simulink model "Engine_Plant_Live"  (R2026b)
settings: Solver=ode1  StartTime=0  StopTime=simcfg.stop_time  FixedStep=0.001
undefined symbols (not defined in the file): constants, ident, init, limits, simcfg
settings Model: Creator=leont  LastModifiedBy=williamvandevoir
settings DataIOCC: ExternalInput=data.ext_in  SaveOutput=off

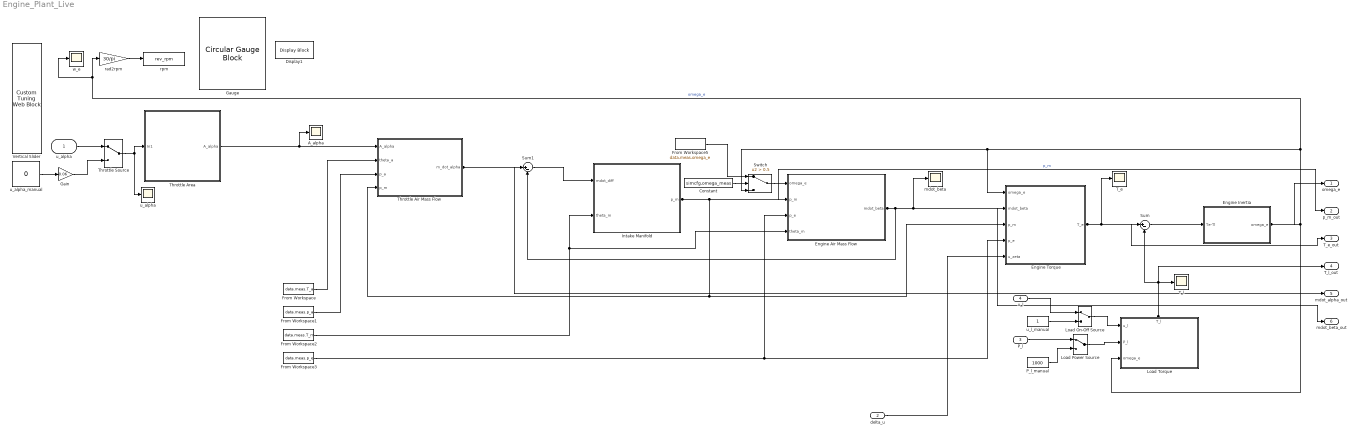
== system Engine_Plant_Live ==
  u_alpha : Inport
  delta_u : Inport  Port=2
  P_l : Inport  Port=3
  u_l : Inport  Port=4
  A_alpha : Scope
      settings: DataLoggingVariableName=ScopeData4
  Constant : Constant  Value=simcfg.omega_meas
  Display1 : DisplayBlock  LabelPosition=Hide  Format=Integer  Transparency=1  GridColor=[0.502, 0.502, 0.502]
  Engine Air Mass Flow : Subsystem
  Engine Inertia : Subsystem
  Engine Torque : Subsystem
  From Workspace : FromWorkspace  VariableName=data.meas.T_a
  From Workspace1 : FromWorkspace  VariableName=data.meas.p_a
  From Workspace2 : FromWorkspace  VariableName=data.meas.T_m
  From Workspace3 : FromWorkspace  VariableName=data.meas.p_e
  From Workspace5 : FromWorkspace  VariableName=data.meas.omega_e
  Gain : Gain  Gain=0.06
  Gauge : CircularGaugeBlock  ScaleMax=5000  FontColor=[0.0, 0.0, 0.0]
  Intake Manifold : Subsystem  Description=Adapted from Intake Manifold Exercise (pressure dynamics only): dp_m/dt = R*theta_m/Vm*(mdot_alpha - mdot_beta). One state; theta_m is an input; R instead of kappa*R.
  Load On-Off Source : ManualSwitch
  Load Power Source : ManualSwitch
  Load Torque : Subsystem
      settings: PortSchema="{\"entries\":[{\"content\":{\"sides\":[{\"content\":{\"connectorIds\":[\"In1\",\"In2\",\"In3\"]},\"type\":\"ConnectorPlacement.EquallySpacedRectSide\",\"uuid\":\"10634893-d67a-46d0-98c2-3f8faa6507dc\"},{\"content\":{\"side\":\"RIGHT\"},\"type\":\"ConnectorPlacement.EquallySpacedRectSide\",\"uuid\":\"a9acb188-8b21-47a2-8013-48c002daa6a2\"},{\"content\":{\"connectorIds\":[\"Out1\"],\"side\":\"TOP\"},\"type\":\"ConnectorPlacement.EquallySpacedRectSide\",\"uuid\":\"c0cacd4e-ae12-4b4a-9868-6a43ffe5219b\"}]},\"type\":\"ConnectorPlacement.EquallySpacedConnector\",\"uuid\":\"1dbc25fc-6040-4af1-8208-de8f0fac67f2\"}],\"packageUris\":[\"http://schema.mathworks.com/mf0/Connector/R2020b\"],\"version\":\"1.0\"}"
  P_l_manual : Constant  Value=1000
  Sum : Sum  Inputs=|+-
  Sum1 : Sum  Inputs=|+-
  Switch : Switch  Criteria=u2 > Threshold  Threshold=0.5  SaturateOnIntegerOverflow=off  InputSameDT=off
  T_e : Scope
      settings: ActiveDisplayYMinimum=-24.090812904473726  ActiveDisplayYMaximum=17.370443961385767
  T_l : Scope
      settings: ActiveDisplayYMinimum=61.428571428571431  ActiveDisplayYMaximum=81.428571428571431
  Throttle Air Mass Flow : Subsystem
  Throttle Area : Subsystem
  Throttle Source : ManualSwitch
  Vertical Slider : CustomTuningWebBlock  LabelPosition=Hide  ShowInitialText=on  Configuration="{\"components\":[{\"name\":\"LinearScaleComponent\",\"settings\":{\"bounds\":{\"max\":100,\"min\":0,\"tickInterval\":\"auto\"},\"internalTickHeightScaleFactor\":0.5,\"labelColor\":[255,255,200],\"labelFont\":{\"font\":\"Arial\",\"fontSize\":12},\"labelOffset\":0.05,\"labelTransparency\":1,\"needleImage\":{\"size\":[596,842],\"src\":\"data:image\\/svg+xml;base64,PD94bWwgdmVyc2lvbj0iMS4wIiBlbmNvZGluZz0idXRmLTgiPz4NCjwhLS0gR2VuZXJhdG9yOiBBZG9iZSBJbGx1c3RyYXRvciAyNS4wLjAsIFNWRyBFeHBvcnQgUGx1Zy1JbiAuIFNWRyBWZXJzaW9uOiA2LjAwIEJ1aWxkIDApICAtLT4NCjxzdmcgdmVyc2lvbj0iMS4xIg0KCSBpZD0ic3ZnOCIgeG1sbnM6Y2M9Imh0dHA6Ly9jcmVhdGl2ZWNvbW1vbnMub3JnL25zIyIgeG1sbnM6ZGM9Imh0dHA6Ly9wdXJsLm9yZy9kYy9lbGVtZW50cy8xLjEvIiB4bWxuczppbmtzY2FwZT0iaHR0cDovL3d3dy5pbmtzY2FwZS5vcmcvbmFtZXNw ...(+2420 chars)\",\"srcOrientation\":\"horizontal\"},\"needleOffset\":[0.0642123287671233,-0.8044596912521441],\"needleSize\":{\"height\":0.07668067226890757,\"width\":0.4337797619047619},\"position\":[0.03623949579831933,0.2829861111111111,0.6088789682539683,0.9196428571428571],\"referencePoint\":\"auto\",\"scaleColors\":[],\"scaleColorsSize\":0.2,\"scaleDirection\":\"BT\",\"showLabels\":1,\"showMinorTicks\":0,\"showSpanLine\":1,\"showTicks\":1,\"tickColor\":[252,252,197],\"tickTransparency\":1,\"valueBarColor\":[0,114,189],\"valueBarOffset\":-0.27,\"valueBarSize\":0.1,\"valueBarTransparency\":1}},{\"name\":\"BackgroundImageComponent\",\"settings\":{\"image\":{\"size\":[380,101],\"src\":\"data:image\\/svg+xml;base64,PHN2ZyB4bWxucz0iaHR0cDovL3d3dy53My5vcmcvMjAwMC9zdmciIHhtbG5zOnhsaW5rPSJodHRwOi8vd3d3LnczLm9yZy8xOTk5L3hsaW5rIiB2aWV3Qm94PSIwIDAgMzgwIDEwMSI+PGRlZnM+PHN0eWxlPi5jbHMtMXtmaWxsOiMwMDJiNDI7fS5jbHMtMntmaWxsOiM0MjcwODI7fS5jbHMtM3tmaWxsOnVybCgjcmFkaWFsLWdyYWRpZW50KTt9LmNscy00e2ZpbGw6I2M4YzhjODtzdHJva2U6IzAwMDt9PC9zdHlsZT48cmFkaWFsR3JhZGllbnQgaWQ9InJhZGlhbC1ncmFkaWVudCIgY3g9IjE5MCIgY3k9IjUwLjUiIHI9IjI2OS4yMSIgZ3JhZGllbnRVbml0cz0idXNlclNwYWNlT25Vc2UiPjxzdG9wIG9mZnNldD0iMC4wMSIgc3RvcC1jb2xvcj0iIzNlNGY1OCIvPjxzdG9wIG9mZnNldD0iMC4wNiIgc3RvcC1jb2xvcj0iIzQ0NTc2MSIvPjxzdG9wIG9mZnNldD0iMC4xNSIgc3RvcC1jb2xvcj0iIzU1NmE3NiIvPjxzdG9wIG9mZnNldD0iMC4yNSIgc3RvcC1jb2xvcj0iIzZkODg5NSIvPjxzdG9wIG9mZnNldD0iMC4zOCIgc3RvcC1jb2xvcj0iIzhmYjJjMyIvPjxzdG9wIG9mZnNldD0iMC41MiIgc3RvcC1jb2xvcj0iI2I2ZTRmYSIvPjxzdG9wIG9mZnNldD0iMSIgc3RvcC1jb2xvcj0iIzE1NDY1NyIvPjwvcmFkaWFsR3JhZGllbnQ+PC9kZWZzPjxnIGlkPSJmcmFtZSI+PGcgaWQ9IkxheWVyXzIiIGRhdGEtbmFtZT0iTGF5ZXIgMiI+PGcgaWQ9IkxheWVyXzEtMiIgZGF0YS1uYW1lPSJMYXllciAxLTIiPjxyZWN0IGlkPSJyZWN0MTAzNiIgY2xhc3M9ImNscy0xIiB4PSIxMSIgeT0iMTEiIHdpZHRoPSIzNTgiIGhlaWdodD0iNzkiLz48cGF0aCBpZD0icGF0aDEwMzgiIGNsYXNzPSJjbHMtMiIgZD0iTTgsOFY5M0gzNzJWOFpNMzY5LDkwSDExVjExSDM2OVoiLz48cGF0aCBpZD0icGF0aDEwNDAiIGNsYXNzPSJjbHMtMyIgZD0iTTAsMFYxMDFIMzgwVjBaTTM3Miw5M0g4VjhIMzcyWiIvPjwvZz48L2c+PC9nPjxnIGlkPSJ0cmFjayI+PHBhdGggaWQ9InJlY3QxNjExIiBjbGFzcz0iY2xzLTQiIGQ9Ik0zMy4zNywyNi41OUgzNDYuNjNjNCwwLDcuMjUsMi42LDcuMjUsNS44MWgwYzAsMy4yMS0zLjI1LDUuODItNy4yNSw1LjgySDMzLjM3Yy00LDAtNy4yNS0yLjYxLTcuMjUtNS44MmgwQzI2LjEyLDI5LjE5LDI5LjM3LDI2LjU5LDMzLjM3LDI2LjU5WiIvPjwvZz48L3N2Zz4=\",\"srcOrientation\":\"horizontal\"},\"position\":[0,0,1,1],\"scaleMode\":\"0\"}},{\"name\":\"ForegroundImageComponent\",\"settings\":{\"image\":{\"size\":[0,0],\"src\":\"default\",\"srcOrientation\":[]},\"isForeground\":1,\"position\":[0,0,1,1],\"scaleMode\":\"0\"}}],\"derived\":{\"blockParameters\":{\"ForegroundColor\":[0.9882352941176471,0.9882352941176471,0.7725490196078432],\"Limits\":{\"Max\":100,\"Min\":0,\"Ticks\":\"auto\"},\"ScaleColors\":[],\"ScaleDirection\":\"Clockwise\",\"ScaleMax\":100,\"ScaleMin\":0,\"TickInterval\":\"auto\",\"fixedAspectRatio\":\"on\"}},\"settings\":{\"BindingType\":\"param\",\"aspectRatio\":3.7777777777777777,\"backgroundColor\":[0,0,0,\"1\"],\"backgroundOffset\":0,\"backgroundOpacity\":1,\"fixedAspectRatio\":\"on\",\"foregroundColor\":[252,252,196],\"orientation\":\"vertical\",\"showBackgroundColor\":false,\"value\":0,\"version\":\"R2026b\"},\"type\":\"Slider\"}"
  mdot_beta : Scope
      settings: ActiveDisplayYMinimum=0.0018042416431033796  ActiveDisplayYMaximum=0.0055634535738285336  DataLoggingVariableName=ScopeData2
  rad2rpm : Gain  Gain=30/pi
  rpm : ToWorkspace  VariableName=rev_rpm  SaveFormat=Timeseries  SampleTime=-1
  "u_alpha " : Scope
      settings: DataLoggingVariableName=ScopeData5
  u_alpha_manual : Constant  Value=0
  u_l_manual : Constant
  w_e : Scope
      settings: DataLoggingVariableName=ScopeData3
  omega_e : Outport
  p_m_out : Outport  Port=2
  T_e_out : Outport  Port=3
  T_l_out : Outport  Port=4
  mdot_alpha_out : Outport  Port=5
  mdot_beta_out : Outport  Port=6
  wires:
  Engine Torque/1(T_e) -> Sum/1, T_e/1, T_e_out/1
  delta_u/1 -> Engine Torque/5(u_zeta)
  Engine Inertia/1(omega_e) -> Switch/3, Engine Torque/1(omega_e), rad2rpm/1, w_e/1, Load Torque/3(omega_e), omega_e/1  "omega_e"
  Sum/1 -> Engine Inertia/1(Te-Tl)
  Load Torque/1(T_l) -> Sum/2, T_l/1, T_l_out/1
  Engine Air Mass Flow/1(mdot_beta) -> Sum1/2, mdot_beta/1, Engine Torque/2(mdot_beta), mdot_beta_out/1
  Intake Manifold/1(p_m) -> Engine Torque/3(p_m), Throttle Air Mass Flow/4(p_m), Engine Air Mass Flow/2(p_m), p_m_out/1  "p_m"
  Throttle Air Mass Flow/1(m_dot_alpha) -> Sum1/1, mdot_alpha_out/1
  Sum1/1 -> Intake Manifold/1(mdot_diff)
  Throttle Area/1(A_alpha) -> A_alpha/1, Throttle Air Mass Flow/1(A_alpha)
  From Workspace1/1 -> Throttle Air Mass Flow/3(p_a)
  From Workspace/1 -> Throttle Air Mass Flow/2(theta_a)
  From Workspace3/1 -> Engine Torque/4(p_e), Engine Air Mass Flow/3(p_e)
  From Workspace2/1 -> Intake Manifold/2(theta_m), Engine Air Mass Flow/4(theta_m)
  u_alpha/1 -> Throttle Source/1
  u_alpha_manual/1 -> Gain/1
  Throttle Source/1 -> "u_alpha "/1, Throttle Area/1(In1)
  Gain/1 -> Throttle Source/2
  u_l_manual/1 -> Load On-Off Source/2
  Load On-Off Source/1 -> Load Torque/1(u_l)
  P_l_manual/1 -> Load Power Source/2
  Load Power Source/1 -> Load Torque/2(P_l)
  rad2rpm/1 -> rpm/1
  Switch/1 -> Engine Air Mass Flow/1(omega_e)
  From Workspace5/1 -> Switch/1
  Constant/1 -> Switch/2
  P_l/1 -> Load Power Source/1
  u_l/1 -> Load On-Off Source/1

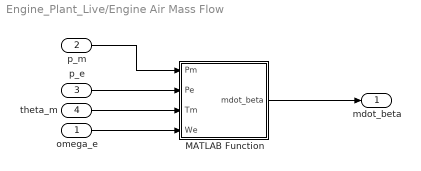
== system Engine_Plant_Live/Engine Air Mass Flow ==
  omega_e : Inport
  p_m : Inport  Port=2
  p_e : Inport  Port=3
  theta_m : Inport  Port=4
  MATLAB Function : MATLAB Function  TreatAsAtomicUnit=on
  mdot_beta : Outport
  wires:
  p_e/1 -> MATLAB Function/2(Pe)
  theta_m/1 -> MATLAB Function/3(Tm)
  omega_e/1 -> MATLAB Function/4(We)
  MATLAB Function/1(mdot_beta) -> mdot_beta/1
  p_m/1 -> MATLAB Function/1(Pm)

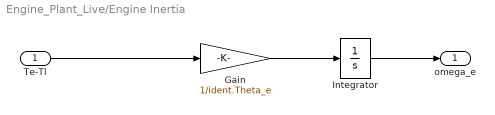
== system Engine_Plant_Live/Engine Inertia ==
  Te-Tl : Inport
  Gain : Gain  Gain=1/ident.Theta_e
  Integrator : Integrator  InitialCondition=init.omega_e0  LimitOutput=on  UpperSaturationLimit=limits.w_max  LowerSaturationLimit=limits.w_min
  omega_e : Outport
  wires:
  Gain/1 -> Integrator/1
  Integrator/1 -> omega_e/1
  Te-Tl/1 -> Gain/1

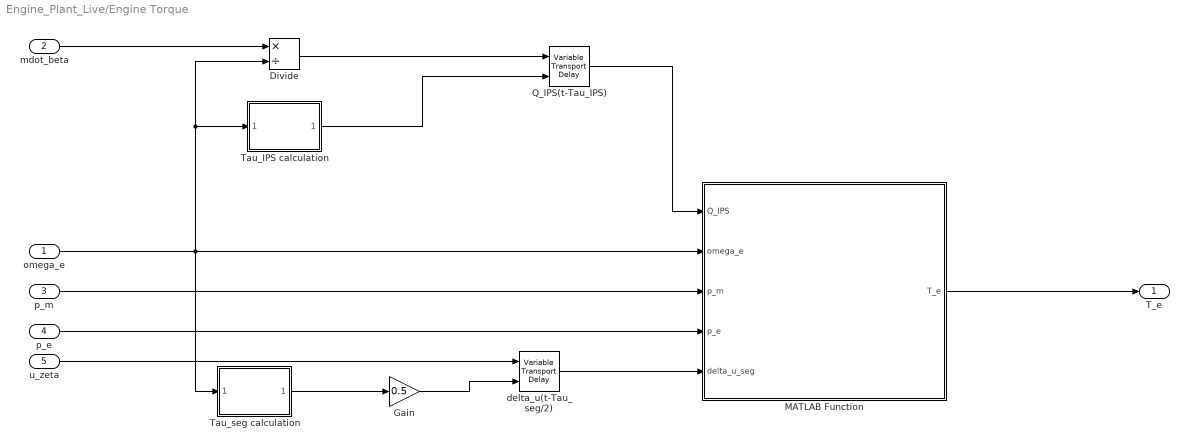
== system Engine_Plant_Live/Engine Torque ==
  omega_e : Inport
  mdot_beta : Inport  Port=2
  p_m : Inport  Port=3
  p_e : Inport  Port=4
  u_zeta : Inport  Port=5
  Divide : Product  Inputs=*/
  Gain : Gain  Gain=0.5
  MATLAB Function : MATLAB Function  TreatAsAtomicUnit=on
  Q_IPS(t-Tau_IPS) : VariableTransportDelay  MaximumDelay=limits.tau_max  InitialOutput=init.q_init
  Tau_IPS calculation : MATLAB Function  TreatAsAtomicUnit=on
  Tau_seg calculation : MATLAB Function  TreatAsAtomicUnit=on
  delta_u(t-Tau_seg/2) : VariableTransportDelay  MaximumDelay=limits.tau_max  InitialOutput=init.du_init
  T_e : Outport
  wires:
  Gain/1 -> delta_u(t-Tau_seg/2)/2
  p_m/1 -> MATLAB Function/3(p_m)
  omega_e/1 -> Divide/2, Tau_IPS calculation/1(omega_e), Tau_seg calculation/1(omega_e), MATLAB Function/2(omega_e)
  Q_IPS(t-Tau_IPS)/1 -> MATLAB Function/1(Q_IPS)
  Tau_IPS calculation/1(Tau_IPS) -> Q_IPS(t-Tau_IPS)/2
  Tau_seg calculation/1(Tau_seg) -> Gain/1
  delta_u(t-Tau_seg/2)/1 -> MATLAB Function/5(delta_u_seg)
  u_zeta/1 -> delta_u(t-Tau_seg/2)/1
  MATLAB Function/1(T_e) -> T_e/1
  p_e/1 -> MATLAB Function/4(p_e)
  Divide/1 -> Q_IPS(t-Tau_IPS)/1
  mdot_beta/1 -> Divide/1

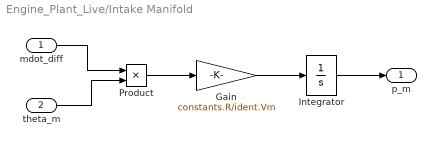
== system Engine_Plant_Live/Intake Manifold ==
  mdot_diff : Inport
  theta_m : Inport  Port=2
  Gain : Gain  Gain=constants.R/ident.Vm
  Integrator : Integrator  InitialCondition=init.p_m0
  Product : Product
  p_m : Outport
  wires:
  mdot_diff/1 -> Product/1
  theta_m/1 -> Product/2
  Product/1 -> Gain/1
  Gain/1 -> Integrator/1
  Integrator/1 -> p_m/1

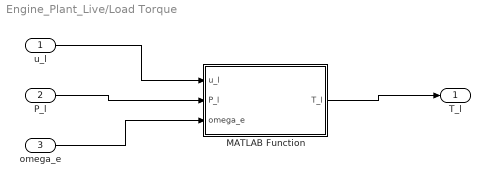
== system Engine_Plant_Live/Load Torque ==
  u_l : Inport
  P_l : Inport  Port=2
  omega_e : Inport  Port=3
  MATLAB Function : MATLAB Function  TreatAsAtomicUnit=on
  T_l : Outport
  wires:
  u_l/1 -> MATLAB Function/1(u_l)
  P_l/1 -> MATLAB Function/2(P_l)
  omega_e/1 -> MATLAB Function/3(omega_e)
  MATLAB Function/1(T_l) -> T_l/1

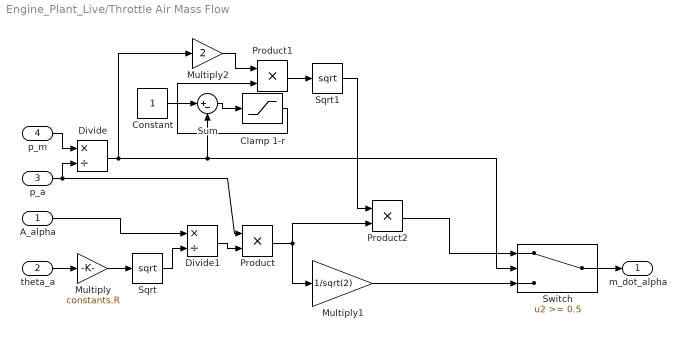
== system Engine_Plant_Live/Throttle Air Mass Flow ==
  A_alpha : Inport
  theta_a : Inport  Port=2
  p_a : Inport  Port=3
  p_m : Inport  Port=4
  Clamp 1-r : Saturate  UpperLimit=inf  LowerLimit=0
  Constant : Constant
  Divide : Product  Inputs=*/
  Divide1 : Product  Inputs=*/
  Multiply : Gain  Gain=constants.R
  Multiply1 : Gain  Gain=1/sqrt(2)
  Multiply2 : Gain  Gain=2
  Product : Product
  Product1 : Product
  Product2 : Product
  Sqrt : Sqrt
  Sqrt1 : Sqrt
  Sum : Sum  Inputs=|+-
  Switch : Switch  Threshold=0.5  SaturateOnIntegerOverflow=off  InputSameDT=off
  m_dot_alpha : Outport
  wires:
  Multiply/1 -> Sqrt/1
  Multiply2/1 -> Product1/1
  Divide/1 -> Switch/2, Sum/2, Multiply2/1
  A_alpha/1 -> Divide1/1
  p_m/1 -> Divide/1
  Divide1/1 -> Product/2
  Product/1 -> Product2/2, Multiply1/1
  Constant/1 -> Sum/1
  Switch/1 -> m_dot_alpha/1
  theta_a/1 -> Multiply/1
  Multiply1/1 -> Switch/3
  Sqrt1/1 -> Product2/1
  Sqrt/1 -> Divide1/2
  Product1/1 -> Sqrt1/1
  p_a/1 -> Product/1, Divide/2
  Product2/1 -> Switch/1
  Sum/1 -> Clamp 1-r/1
  Clamp 1-r/1 -> Product1/2

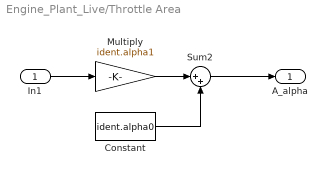
== system Engine_Plant_Live/Throttle Area ==
  In1 : Inport
  Constant : Constant  Value=ident.alpha0
  Multiply : Gain  Gain=ident.alpha1
  Sum2 : Sum  Inputs=|++
  A_alpha : Outport
  wires:
  Multiply/1 -> Sum2/1
  Constant/1 -> Sum2/2
  In1/1 -> Multiply/1
  Sum2/1 -> A_alpha/1

== matlab function Engine_Plant_Live/Engine Torque/Tau_IPS calculation ==
  data: omega_e input; Tau_IPS output
function Tau_IPS = fcn(omega_e)

    if omega_e > 0
        Tau_IPS = 2*pi/omega_e;
    
    else
        Tau_IPS = 0;
    end

end

== matlab function Engine_Plant_Live/Engine Torque/MATLAB Function ==
  data: Q_IPS input; omega_e input; p_m input; p_e input; delta_u_seg input; T_e output size=1; ident parameter; constants parameter
function T_e = fcn(Q_IPS, omega_e, p_m, p_e, delta_u_seg, ident, constants)

%% Parameters to identify: beta0, eta0, eta1

p_me0f = ident.beta0 * 4*pi/constants.Vd;
p_me0g = p_e - p_m;
e_zeta = 1 - constants.k_zeta*(delta_u_seg^2);
ep_mphi = (ident.eta0 + ident.eta1*omega_e)*e_zeta*constants.Hl*4*pi*Q_IPS/(constants.Vd*constants.lambda*constants.sigma0);

p_me = (ep_mphi - p_me0f - p_me0g);


T_e = p_me*constants.Vd/(4*pi);

== matlab function Engine_Plant_Live/Engine Torque/Tau_seg calculation ==
  data: omega_e input; Tau_seg output
function Tau_seg = fcn(omega_e)

    if omega_e > 0
        Tau_seg = 4*pi/(5*omega_e);
    
    else
        Tau_seg = 0;
    end

end

== matlab function Engine_Plant_Live/Load Torque/MATLAB Function ==
  data: u_l input; T_l output size=1; P_l input; omega_e input; constants parameter
function T_l = fcn(u_l, P_l, omega_e, constants)
% Load torque: T_l = u_l * P_l / (omega_e * eta_gen)
% u_l: load on/off (1/0), P_l: load power [W], omega_e: engine speed [rad/s]
T_l = u_l * P_l / (omega_e * constants.eta_gen);

== matlab function Engine_Plant_Live/Engine Air Mass Flow/MATLAB Function ==
  data: Pm input; mdot_beta output size=1; Pe input; Tm input; We input; constants parameter; ident parameter
function mdot_beta = fcn(Pm, Pe, Tm, We, constants, ident)
% Engine Air Mass Flow: air mass flow leaving the intake manifold [kg/s]
% Inputs: Pm [Pa], Pe [Pa], Tm [K], We [rad/s]

% volumetric efficiency, pressure part (residual gas, polytropic expansion)
lam_lp = (constants.Vc + constants.Vd)/constants.Vd - (constants.Vc/constants.Vd) * (max(Pe/Pm, 0))^(1/constants.kappa);

% volumetric efficiency, speed part (linear in We, identified in milestone 2)
lam_lw = ident.gamma0 + ident.gamma1*We;

% air mass flow into the engine (four-stroke engine: factor 1/2)
mdot_e = 0.5 * Pm/(constants.R*Tm) * (lam_lp*lam_lw) * constants.Vd * We/(2*pi);

% air mass flow from the manifold (the rest is fuel, ratio lambda*sigma0)
mdot_beta = mdot_e / (1 + 1/(constants.lambda*constants.sigma0));
